simulink subsystem "PowerSplitDriveUnit_refsub_Basic"  (R2023a)
settings: Solver=VariableStepAuto  StartTime=0.0  StopTime=10.0  RelTol=1e-3
undefined symbols (not defined in the file or in its folder): initial, motorGenerator1, motorGenerator2
settings Model: Creator=isaacito  LastModifiedBy=isaacito
settings SolverCC: AlgebraicLoopSolver=TrustRegion
settings OptimizationCC: ReuseModelBlockBuffer=off
settings DebuggingCC: UnconnectedInputMsg=warning  UnconnectedOutputMsg=warning  UnconnectedLineMsg=warning
settings ModelReferenceCC: EnableRefExpFcnMdlSchedulingChecks=on
settings RTWCC: DLArmComputeVersion=19.05

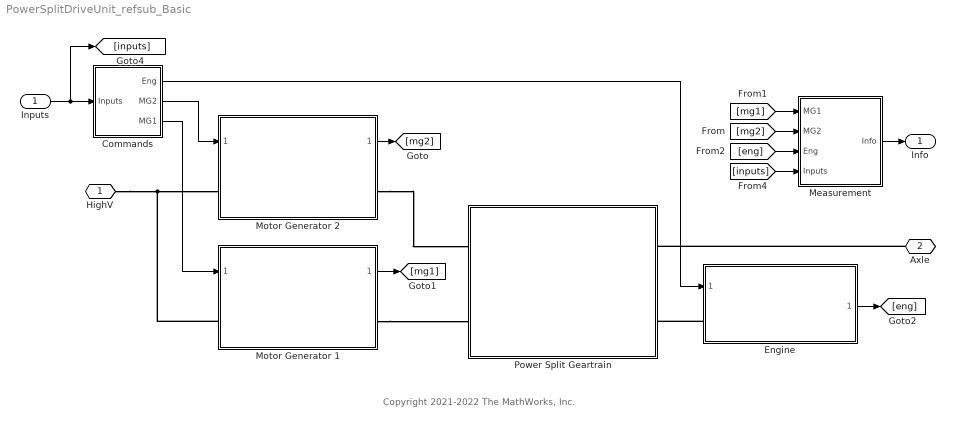
== system PowerSplitDriveUnit_refsub_Basic ==
  note: Copyright 2021-2022 The MathWorks, Inc.
  Inputs : Inport
  Commands : Subsystem
  Engine : Subsystem  ReferencedSubsystem=Engine_refsub_Basic
  Measurement : Subsystem
  Motor Generator 1 : Subsystem  ReferencedSubsystem=MotorDriveUnit_refsub_Basic  torque_max=motorGenerator1.trqMax_Nm  Value=motorGenerator1.powerMax_kW  Tc=motorGenerator1.responseTime_s  eff=motorGenerator1.efficiency_pct  w_eff=motorGenerator1.spd_eff_rpm  T_eff=motorGenerator1.trq_eff_Nm  thermal_mass=motorGenerator1.thermalMass_J_perK  temperature=initial.MG1_Temperature_K  k=motorGenerator1.dampSpringStiffness_Nm_per_rad  mu_visc=motorGenerator1.dampSpringFriction_Nm_per_rpm  w_tol=smoothing.MG1_dampSpringVelTol_rpm  T=initial.MG1_AirTemp_K
      settings: PortSchema="{\"entries\":[{\"content\":{\"sides\":[{\"content\":{\"connectorIds\":[\"In1\",\"LConn1\"]},\"type\":\"ConnectorPlacement.EquallySpacedRectSide\",\"uuid\":\"02d16a10-ccfb-4288-a5a1-1144159c5ca2\"},{\"content\":{\"connectorIds\":[\"Out1\",\"LConn2\"],\"side\":\"RIGHT\"},\"type\":\"ConnectorPlacement.EquallySpacedRectSide\",\"uuid\":\"b2601986-efe5-4f5e-bd54-3f5cb03e9252\"},{\"content\":{\"connectorIds\":[],\"side\":\"TOP\"},\"type\":\"ConnectorPlacement.EquallySpacedRectSide\",\"uuid\":\"248805f0-4416-4f49-8b0b-c2d3fe77e89e\"}]},\"type\":\"ConnectorPlacement.EquallySpacedConnector\",\"uuid\":\"35449164-35fe-478e-9b2e-66e853caa6da\"}],\"packageUris\":[\"http://schema.mathworks.com/mf0/Connector/R2020b\"],\"version\":\"1.0\"}"
  Motor Generator 2 : Subsystem  ReferencedSubsystem=MotorDriveUnit_refsub_Basic  torque_max=motorGenerator2.trqMax_Nm  Value=motorGenerator2.powerMax_kW  Tc=motorGenerator2.responseTime_s  eff=motorGenerator2.efficiency_pct  w_eff=motorGenerator2.spd_eff_rpm  T_eff=motorGenerator2.trq_eff_Nm  thermal_mass=motorGenerator2.thermalMass_J_perK  temperature=initial.MG2_Temperature_K  k=motorGenerator2.dampSpringStiffness_Nm_per_rad  mu_visc=motorGenerator2.dampSpringFriction_Nm_per_rpm  w_tol=smoothing.MG2_dampSpringVelTol_rpm  T=initial.MG2_AirTemp_K
      settings: PortSchema="{\"entries\":[{\"content\":{\"sides\":[{\"content\":{\"connectorIds\":[\"In1\",\"LConn1\"]},\"type\":\"ConnectorPlacement.EquallySpacedRectSide\",\"uuid\":\"02d16a10-ccfb-4288-a5a1-1144159c5ca2\"},{\"content\":{\"connectorIds\":[\"Out1\",\"LConn2\"],\"side\":\"RIGHT\"},\"type\":\"ConnectorPlacement.EquallySpacedRectSide\",\"uuid\":\"b2601986-efe5-4f5e-bd54-3f5cb03e9252\"},{\"content\":{\"connectorIds\":[],\"side\":\"TOP\"},\"type\":\"ConnectorPlacement.EquallySpacedRectSide\",\"uuid\":\"248805f0-4416-4f49-8b0b-c2d3fe77e89e\"}]},\"type\":\"ConnectorPlacement.EquallySpacedConnector\",\"uuid\":\"35449164-35fe-478e-9b2e-66e853caa6da\"}],\"packageUris\":[\"http://schema.mathworks.com/mf0/Connector/R2020b\"],\"version\":\"1.0\"}"
  Power Split Geartrain : Subsystem  ReferencedSubsystem=PowerSplitGeartrain_refsub_Basic
      settings: PortSchema="{\"entries\":[{\"content\":{\"sides\":[{\"content\":{\"connectorIds\":[\"LConn3\",\"LConn2\"]},\"type\":\"ConnectorPlacement.EquallySpacedRectSide\",\"uuid\":\"39b05f33-5a15-4788-a57f-d6050162e484\"},{\"content\":{\"connectorIds\":[\"LConn1\",\"LConn4\"],\"side\":\"RIGHT\"},\"type\":\"ConnectorPlacement.EquallySpacedRectSide\",\"uuid\":\"22b56448-375b-40fb-9a49-9bd466a0970b\"},{\"content\":{\"connectorIds\":[],\"side\":\"TOP\"},\"type\":\"ConnectorPlacement.EquallySpacedRectSide\",\"uuid\":\"d8d57956-46e4-4991-901b-1ed920cdc976\"}]},\"type\":\"ConnectorPlacement.EquallySpacedConnector\",\"uuid\":\"bf43f8af-bced-41cd-bdc5-a4c4cabcb371\"}],\"packageUris\":[\"http://schema.mathworks.com/mf0/Connector/R2020b\"],\"version\":\"1.0\"}"
  HighV : PMIOPort  Side=Left
  Axle : PMIOPort  Port=2  Side=Right
  Info : Outport
  wires:
  Motor Generator 2/1 -> [mg2]
  [mg2] -> Measurement/2(MG2)
  [mg1] -> Measurement/1(MG1)
  [eng] -> Measurement/3(Eng)
  [inputs] -> Measurement/4(Inputs)
  Measurement/1(Info) -> Info/1
  Motor Generator 1/1 -> [mg1]
  Engine/1 -> [eng]
  Inputs/1 -> Commands/1(Inputs), [inputs]
  Commands/2(MG2) -> Motor Generator 2/1
  Commands/3(MG1) -> Motor Generator 1/1
  Commands/1(Eng) -> Engine/1
  connections:
  HighV/RConn1 -- Motor Generator 1/LConn1 -- Motor Generator 2/LConn1
  Engine/LConn1 -- Power Split Geartrain/LConn4
  Axle/RConn1 -- Power Split Geartrain/LConn1
  Motor Generator 2/LConn2 -- Power Split Geartrain/LConn3
  Motor Generator 1/LConn2 -- Power Split Geartrain/LConn2

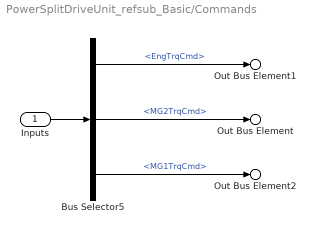
== system PowerSplitDriveUnit_refsub_Basic/Commands ==
  Inputs : Inport
  Bus Selector5 : BusSelector  OutputSignals=EngTrqCmd,MG2TrqCmd,MG1TrqCmd
  Out Bus Element1 : Outport  PortName=Eng  Element=TrqCmd
  Out Bus Element : Outport  Port=2  PortName=MG2  Element=TrqCmd
  Out Bus Element2 : Outport  Port=3  PortName=MG1  Element=TrqCmd
  wires:
  Bus Selector5/1 -> Out Bus Element1/1  "<EngTrqCmd>"
  Bus Selector5/3 -> Out Bus Element2/1  "<MG1TrqCmd>"
  Bus Selector5/2 -> Out Bus Element/1  "<MG2TrqCmd>"
  Inputs/1 -> Bus Selector5/1

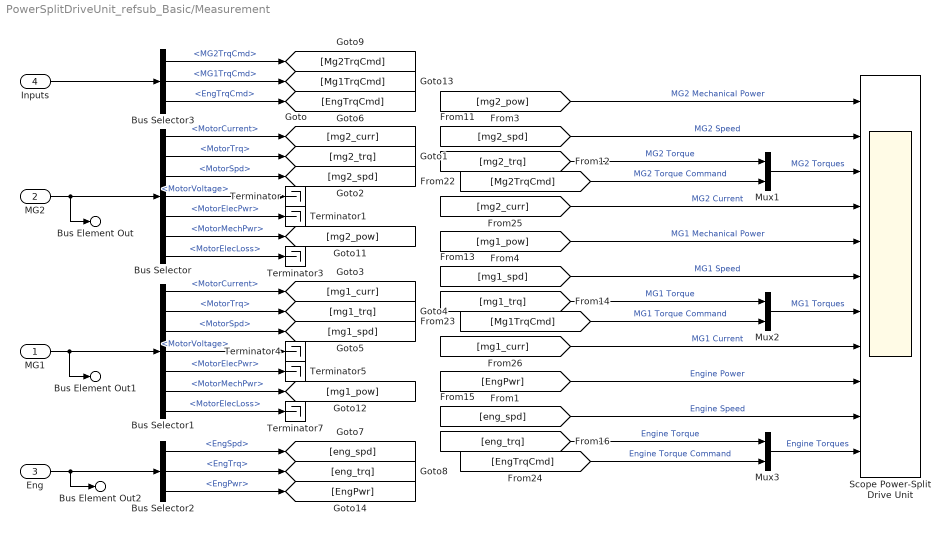
== system PowerSplitDriveUnit_refsub_Basic/Measurement ==
  MG1 : Inport
  MG2 : Inport  Port=2
  Eng : Inport  Port=3
  Inputs : Inport  Port=4
  Bus Selector : BusSelector  OutputSignals=MotorCurrent,MotorTrq,MotorSpd,MotorVoltage,MotorElecPwr,MotorMechPwr,MotorElecLoss
  Bus Selector1 : BusSelector  OutputSignals=MotorCurrent,MotorTrq,MotorSpd,MotorVoltage,MotorElecPwr,MotorMechPwr,MotorElecLoss
  Bus Selector2 : BusSelector  OutputSignals=EngSpd,EngTrq,EngPwr
  Bus Selector3 : BusSelector  OutputSignals=MG2TrqCmd,MG1TrqCmd,EngTrqCmd
  Mux1 : Mux  Inputs=2
  Mux2 : Mux  Inputs=2
  Mux3 : Mux  Inputs=2
  Scope Power-Split Drive Unit : Scope  NumInputPorts=11
  Terminator{,1,3..5,7} (6 alike) : Terminator
  Bus Element Out2 : Outport  PortName=Info  Element=eng
  Bus Element Out : Outport  PortName=Info  Element=mg2
  Bus Element Out1 : Outport  PortName=Info  Element=mg1
  wires:
  [EngPwr] -> Scope Power-Split Drive Unit/9  "Engine Power"
  Bus Selector2/3 -> [EngPwr]  "<EngPwr>"
  [mg2_pow] -> Scope Power-Split Drive Unit/1  "MG2 Mechanical Power"
  [mg1_pow] -> Scope Power-Split Drive Unit/5  "MG1 Mechanical Power"
  Bus Selector1/4 -> Terminator4/1  "<MotorVoltage>"
  Bus Selector1/7 -> Terminator7/1  "<MotorElecLoss>"
  Bus Selector1/6 -> [mg1_pow]  "<MotorMechPwr>"
  Bus Selector1/5 -> Terminator5/1  "<MotorElecPwr>"
  Bus Selector/7 -> Terminator3/1  "<MotorElecLoss>"
  Bus Selector/6 -> [mg2_pow]  "<MotorMechPwr>"
  Bus Selector/5 -> Terminator1/1  "<MotorElecPwr>"
  Bus Selector/4 -> Terminator/1  "<MotorVoltage>"
  Mux3/1 -> Scope Power-Split Drive Unit/11  "Engine Torques"
  [eng_spd] -> Scope Power-Split Drive Unit/10  "Engine Speed"
  [mg1_curr] -> Scope Power-Split Drive Unit/8  "MG1 Current"
  Mux2/1 -> Scope Power-Split Drive Unit/7  "MG1 Torques"
  [mg1_spd] -> Scope Power-Split Drive Unit/6  "MG1 Speed"
  Bus Selector3/3 -> [EngTrqCmd]  "<EngTrqCmd>"
  Bus Selector3/2 -> [Mg1TrqCmd]  "<MG1TrqCmd>"
  Bus Selector3/1 -> [Mg2TrqCmd]  "<MG2TrqCmd>"
  Inputs/1 -> Bus Selector3/1
  Bus Selector2/2 -> [eng_trq]  "<EngTrq>"
  Bus Selector2/1 -> [eng_spd]  "<EngSpd>"
  Bus Selector1/3 -> [mg1_spd]  "<MotorSpd>"
  Bus Selector1/2 -> [mg1_trq]  "<MotorTrq>"
  Bus Selector1/1 -> [mg1_curr]  "<MotorCurrent>"
  Bus Selector/3 -> [mg2_spd]  "<MotorSpd>"
  Bus Selector/2 -> [mg2_trq]  "<MotorTrq>"
  Bus Selector/1 -> [mg2_curr]  "<MotorCurrent>"
  [mg2_spd] -> Scope Power-Split Drive Unit/2  "MG2 Speed"
  [eng_trq] -> Mux3/1  "Engine Torque"
  [mg2_curr] -> Scope Power-Split Drive Unit/4  "MG2 Current"
  [mg1_trq] -> Mux2/1  "MG1 Torque"
  [Mg1TrqCmd] -> Mux2/2  "MG1 Torque Command"
  [Mg2TrqCmd] -> Mux1/2  "MG2 Torque Command"
  Mux1/1 -> Scope Power-Split Drive Unit/3  "MG2 Torques"
  [mg2_trq] -> Mux1/1  "MG2 Torque"
  [EngTrqCmd] -> Mux3/2  "Engine Torque Command"
  Eng/1 -> Bus Selector2/1, Bus Element Out2/1
  MG1/1 -> Bus Element Out1/1, Bus Selector1/1
  MG2/1 -> Bus Element Out/1, Bus Selector/1
